simulink model "open_loop_deploy"  (R2026b)
settings: Solver=FixedStepAuto  StopTime=10  EnableMultiTasking=on
undefined symbols (not defined in the file): Bambient, bits, k, R_coil_ref, Vmax
libraries: stm32blockslib x6, stm32f4xxblockslib x1, simulink x1
settings Model: STM32="{\"PWMOutput\":{\"ID\":\"274\"},\"TimerCapture\":[{\"ID\":\"277\"},{\"ID\":\"278\"},{\"ID\":\"279\"},{\"ID\":\"280\"}],\"UARTRead\":{\"ID\":\"339\"},\"UARTWrite\":[{\"ID\":\"366\"},{\"ID\":\"380\"}],\"I2CControllerRead\":{\"ID\":\"388\"},\"I2CControllerWrite\":[{\"ID\":\"398\"},{\"ID\":\"400\"},{\"ID\":\"401\"}]}"  Creator=Samuel  LastModifiedBy=samue
settings SolverCC: AutoInsertRateTranBlk=on
settings OptimizationCC: DefaultParameterBehavior=Inlined  DifferentSizesBufferReuse=on  EfficientTunableParamExpr=on  EnhancedBackFolding=on  MaxStackSize=512  OptimizationCustomize=off  OptimizeBlockOrder=speed  PassReuseOutputArgsAs=Individual arguments  RemoveInternalMemoryZeroInit=on  RemoveRootLevelIOMemoryZeroInit=on
settings DebuggingCC: ParameterTunabilityLossMsg=error
settings HardwareCC: ProdHWDeviceType=ARM Compatible->ARM Cortex-M  ProdLargestAtomicFloat=Double  ProdLargestAtomicInteger=Long  ProdLongLongMode=on
settings SFSimCC: MATLABDynamicMemAlloc=off
settings RTWCC: BuildConfiguration=Faster Runs  Description=Embedded Coder  HardwareBoard=STM32G4xx Based  SystemTargetFile=ert.tlc  TLCOptions=-aInlineSetEventsForThisBaseRateFcn=TLC_FALSE -aSuppressMultiTaskScheduler=TLC_FALSE -aRateBasedStepFcn=1  TemplateMakefile=ert_default_tmf  Toolchain=GNU Tools for STM32
settings CodeAppCC: ForceParamTrailComments=on  IgnoreCustomStorageClasses=off  InsertBlockDesc=on  OperatorAnnotations=on  SFDataObjDesc=on  SimulinkDataObjDesc=on
settings ERTTargetCC: CodeReplacementLibrary=ARM Cortex-M  CombineSignalStateStructs=on  ExtModeIntrfLevel=Level2 - Open  ExtModeMexFile=ext_xcp  ExtModeStaticAlloc=on  SupportVariableSizeSignals=on
settings SimscapeCC: SimscapeUseEnergyAccounting=off

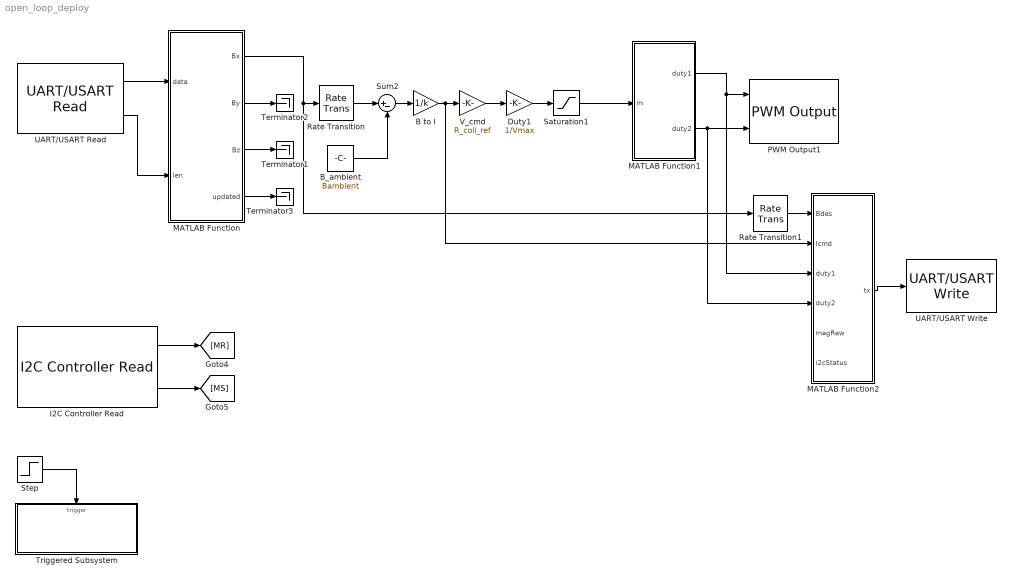
== system open_loop_deploy ==
  B to I : Gain  Gain=1/k
  B_ambient : Constant  Value=Bambient
  Duty1 : Gain  Gain=1/Vmax
  I2C Controller Read : stm32blockslib/I2C Controller Read  I2CModule=I2C1  Mode=Controller  AddressingMode=7-bits  PeripheralByteOrder=BigEndian  OwnPeripheralAddress=uint8(170)  PeripheralAddressVia=Dialog  PeripheralAddress=hex2dec('21')  RegisterAddressMode=on  RegisterAddressVia=Dialog  RegisterAddress=hex2dec('24')  RepeatedStart=off  NoAck=off  OutputStatus=on  BlockMode=Receive  DataType=uint8  DataLength=9  Timeout=0.005  SampleTime=0.01
      settings: LibrarySourceBlock=stm32g4xxblockslib/I2C Controller Read
  MATLAB Function : MATLAB Function  TreatAsAtomicUnit=on
  MATLAB Function1 : MATLAB Function  TreatAsAtomicUnit=on
  MATLAB Function2 : MATLAB Function  TreatAsAtomicUnit=on
  PWM Output1 : stm32f4xxblockslib/PWM Output  ProcessorFamily=STM32G4  TimerModule=TIM1  DutycycleUnits=Percentage  EnableChannel1=on  EnableCaptureCompare1Input=off  EnableCaptureCompare1ComplementaryInput=off  EnableOutputCompare1ModeInput=off  EnableChannel2=on  EnableCaptureCompare2Input=off  EnableCaptureCompare2ComplementaryInput=off  EnableOutputCompare2ModeInput=off  EnableChannel3=off  EnableCaptureCompare3Input=off  EnableCaptureCompare3ComplementaryInput=off  EnableOutputCompare3ModeInput=off  EnableChannel4=off  EnableCaptureCompare4Input=off  EnableCaptureCompare4ComplementaryInput=off  EnableOutputCompare4ModeInput=off  EnableChannel5=off  EnableCaptureCompare5Input=off  EnableOutputCompare5ModeInput=off  EnableChannel6=off  EnableCaptureCompare6Input=off  EnableOutputCompare6ModeInput=off  EnableCounterInput=off  EnableMainOutputInput=off  EnableFrequencyInput=off  SetRCAfterCE=off  OutputDirection=off  OutputMainOutputEnableStatus=off  SampleTime=0.1  EnableSimPort=off  EnableUpdateEvent=off  EnableCaptureCompare1Event=off  EnableCaptureCompare2Event=off  EnableCaptureCompare3Event=off  EnableCaptureCompare4Event=off  EnableTriggerEvent=off  EnableBreakEvent=off  EnableBreakEvent2=off  hoistedMaskSrc=ECSoC/ECSimCodegen/PWM Output
      settings: LibrarySourceBlock=stm32g4xxblockslib/PWM Output
  Rate Transition : RateTransition  OutPortSampleTime=0.1
  Rate Transition1 : RateTransition  OutPortSampleTime=0.1
  Saturation1 : Saturate  UpperLimit=1  LowerLimit=-1
  Step : Step  Time=0.1  SampleTime=0.1
  Sum2 : Sum  Inputs=|+-
  Terminator1 : Terminator
  Terminator2 : Terminator
  Terminator3 : Terminator
  Triggered Subsystem : Subsystem  TreatAsAtomicUnit=on
  UART/USART Read : stm32blockslib/UART//USART Read  UARTModule=LPUART1  DataType=uint8  DataLength=32  BlockingMode=off  BlockingTimeout=0.1  OutputLength=on  OutputStatus=off  SampleTime=0.001
  UART/USART Write : stm32blockslib/UART//USART Write  UARTModule=LPUART1  LengthOfDataToSend=off  BlockingMode=off  BlockingTimeout=0.1  OutputStatus=off
  V_cmd : Gain  Gain=R_coil_ref
  wires:
  B_ambient/1 -> Sum2/2
  Sum2/1 -> B to I/1
  Saturation1/1 -> MATLAB Function1/1(m)
  Duty1/1 -> Saturation1/1
  V_cmd/1 -> Duty1/1
  UART/USART Read/1 -> MATLAB Function/1(data)
  MATLAB Function/3(Bz) -> Terminator1/1
  MATLAB Function/2(By) -> Terminator2/1
  Rate Transition/1 -> Sum2/1
  MATLAB Function/1(Bx) -> Rate Transition/1, Rate Transition1/1
  UART/USART Read/2 -> MATLAB Function/2(len)
  MATLAB Function/4(updated) -> Terminator3/1
  MATLAB Function2/1(tx) -> UART/USART Write/1
  B to I/1 -> MATLAB Function2/2(Icmd), V_cmd/1
  MATLAB Function1/1(duty1) -> MATLAB Function2/3(duty1), PWM Output1/1
  Rate Transition1/1 -> MATLAB Function2/1(Bdes)
  MATLAB Function1/2(duty2) -> MATLAB Function2/4(duty2), PWM Output1/2
  I2C Controller Read/1 -> [MR]
  I2C Controller Read/2 -> [MS]
  Step/1 -> Triggered Subsystem/Trigger

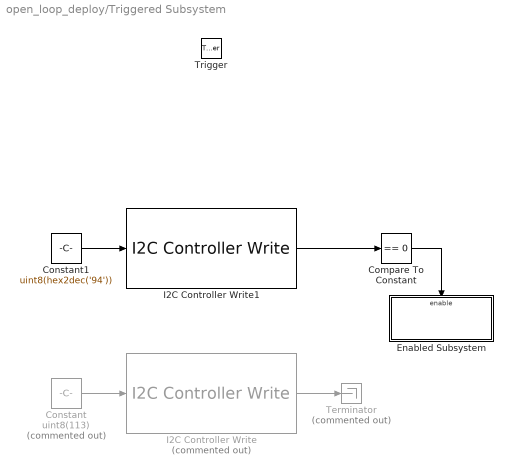
== system open_loop_deploy/Triggered Subsystem ==
  Trigger : TriggerPort  VariantControl=(inherit)
  Compare To Constant : simulink/Logic and Bit Operations/Compare To Constant  relop===  const=0  OutDataTypeStr=boolean
  Constant : Constant  Commented=on  Value=uint8(113)
  Constant1 : Constant  Value=uint8(hex2dec('94'))
  Enabled Subsystem : Subsystem  TreatAsAtomicUnit=on
  I2C Controller Write : stm32blockslib/I2C Controller Write  Commented=on  I2CModule=I2C1  Mode=Controller  AddressingMode=7-bits  PeripheralByteOrder=BigEndian  OwnPeripheralAddress=uint8(170)  PeripheralAddressVia=Dialog  PeripheralAddress=hex2dec('21')  RegisterAddressMode=on  RegisterAddressVia=Dialog  RegisterAddress=1  RepeatedStart=off  NoAck=off  OutputStatus=on  BlockMode=Transmit  DataType=uint8  DataLength=1  Timeout=0.01  SampleTime=-1
      settings: LibrarySourceBlock=stm32g4xxblockslib/I2C Controller Write
  I2C Controller Write1 : stm32blockslib/I2C Controller Write  I2CModule=I2C1  Mode=Controller  AddressingMode=7-bits  PeripheralByteOrder=BigEndian  OwnPeripheralAddress=uint8(170)  PeripheralAddressVia=Dialog  PeripheralAddress=hex2dec('21')  RegisterAddressMode=on  RegisterAddressVia=Dialog  RegisterAddress=hex2dec('0B')  RepeatedStart=off  NoAck=off  OutputStatus=on  BlockMode=Transmit  DataType=uint8  DataLength=1  Timeout=0.01  SampleTime=-1
      settings: LibrarySourceBlock=stm32g4xxblockslib/I2C Controller Write
  Terminator : Terminator  Commented=on
  wires:
  Constant1/1 -> I2C Controller Write1/1
  Compare To Constant/1 -> Enabled Subsystem/Enable
  I2C Controller Write/1 -> Terminator/1
  Constant/1 -> I2C Controller Write/1
  I2C Controller Write1/1 -> Compare To Constant/1

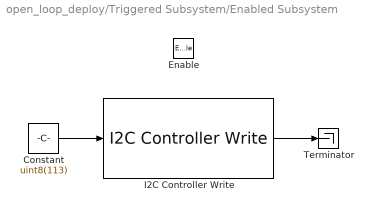
== system open_loop_deploy/Triggered Subsystem/Enabled Subsystem ==
  Enable : EnablePort
  Constant : Constant  Value=uint8(113)
  I2C Controller Write : stm32blockslib/I2C Controller Write  I2CModule=I2C1  Mode=Controller  AddressingMode=7-bits  PeripheralByteOrder=BigEndian  OwnPeripheralAddress=uint8(170)  PeripheralAddressVia=Dialog  PeripheralAddress=hex2dec('21')  RegisterAddressMode=on  RegisterAddressVia=Dialog  RegisterAddress=1  RepeatedStart=off  NoAck=off  OutputStatus=on  BlockMode=Transmit  DataType=uint8  DataLength=1  Timeout=0.01  SampleTime=-1
      settings: LibrarySourceBlock=stm32g4xxblockslib/I2C Controller Write
  Terminator : Terminator
  wires:
  Constant/1 -> I2C Controller Write/1
  I2C Controller Write/1 -> Terminator/1

== matlab function open_loop_deploy/MATLAB Function1 ==
  data: m input; duty1 output; duty2 output
function [duty1, duty2] = drv8871PWM(m)
%#codegen
% m is the normalized voltage command, between -1 and +1.

if m >= 0
    duty1 = 100;
    duty2 = 100 * (1 - m);
else
    duty1 = 100 * (1 + m);
    duty2 = 100;
end

== matlab function open_loop_deploy/MATLAB Function ==
  data: data input; Bx output; len input; By output; Bz output; updated output
function [Bx, By, Bz, updated] = Decode_SET(data, len)
%#codegen
% data: uint8 vector from UART Read, len: number of valid bytes this step.
% GUI sends "SET: x, y, z\n" in microtesla.
persistent buffer count dropping lastB
if isempty(count)
    buffer   = zeros(1, 96, 'uint8');
    count    = 0;
    dropping = false;
    lastB    = zeros(3, 1);
end
updated = false;
nValid = min(double(len), numel(data));
for i = 1:nValid
    b = uint8(data(i));
    if b == 10                          % newline: end of command
        if ~dropping && count > 0
            [vals, ok] = parseSET(buffer, count);
            if ok
                lastB   = vals * 1e-6;  % microtesla -> tesla
                updated = true;
            end
        end
        count    = 0;
        dropping = false;
    elseif b ~= 13                      % ignore carriage return
        if ~dropping
            if count < 96
                count = count + 1;
                buffer(count) = b;
            else
                dropping = true;        % discard oversized line
            end
        end
    end
end
Bx = lastB(1);
By = lastB(2);
Bz = lastB(3);
end

function [vals, ok] = parseSET(buf, n)
vals = zeros(3, 1);
ok = false;
if n < 4
    return;
end
if buf(1) ~= 83 || buf(2) ~= 69 || buf(3) ~= 84 || buf(4) ~= 58   % 'SET:'
    return;
end
pos = 5;
for k = 1:3
    pos = skipSpaces(buf, pos, n);
    if k > 1
        if pos > n || buf(pos) ~= 44    % ','
            return;
        end
        pos = skipSpaces(buf, pos + 1, n);
    end
    [v, pos, good] = parseNum(buf, pos, n);
    if ~good
        return;
    end
    vals(k) = v;
end
pos = skipSpaces(buf, pos, n);
ok = (pos > n);                         % nothing left over
end

function p = skipSpaces(buf, p, n)
while p <= n && (buf(p) == 32 || buf(p) == 9)
    p = p + 1;
end
end

function [v, p, ok] = parseNum(buf, p, n)
v = 0; ok = false; sgn = 1;
if p <= n && (buf(p) == 45 || buf(p) == 43)        % '-' or '+'
    if buf(p) == 45
        sgn = -1;
    end
    p = p + 1;
end
mant = 0; nd = 0;
while p <= n && buf(p) >= 48 && buf(p) <= 57       % integer digits
    mant = mant * 10 + (double(buf(p)) - 48);
    nd = nd + 1; p = p + 1;
end
if p <= n && buf(p) == 46                          % '.'
    p = p + 1; scale = 0.1;
    while p <= n && buf(p) >= 48 && buf(p) <= 57
        mant = mant + (double(buf(p)) - 48) * scale;
        scale = scale / 10;
        nd = nd + 1; p = p + 1;
    end
end
if nd == 0
    return;
end
if p <= n && (buf(p) == 101 || buf(p) == 69)       % 'e' or 'E'
    q = p + 1; esgn = 1;
    if q <= n && (buf(q) == 45 || buf(q) == 43)
        if buf(q) == 45
            esgn = -1;
        end
        q = q + 1;
    end
    ex = 0; ne = 0;
    while q <= n && buf(q) >= 48 && buf(q) <= 57
        ex = ex * 10 + (double(buf(q)) - 48);
        ne = ne + 1; q = q + 1;
    end
    if ne == 0
        return;
    end
    mant = mant * 10^(esgn * ex);
    p = q;
end
v = sgn * mant;
ok = true;
end

== matlab function open_loop_deploy/MATLAB Function2 ==
  data: Bdes input; tx output; Icmd input; duty1 input; duty2 input; magRaw input; i2cStatus input
function tx = Encode_CMD(Bdes, Icmd, duty1, duty2, magRaw, i2cStatus)
%#codegen

values = [double(Bdes)*1e6, double(Icmd), ...
          double(duty1), double(duty2)];

tx = repmat(uint8(32), 1, 80);
tx(1:5) = uint8('CMD: ');
p = 6;

for k = 1:4
    [field, n] = compactNumber(values(k));
    tx(p:p+n-1) = field(1:n);
    p = p + n;
    if k < 4
        tx(p) = uint8(',');
    else
        tx(p) = uint8(10);
    end
    p = p + 1;
end

tx(p:p+4) = uint8('MAG: ');
p = p + 5;

if i2cStatus == 0
    for k = 1:3
        i = 3*(k-1) + 1;
        raw = double(magRaw(i))*65536 ...
            + double(magRaw(i+1))*256 ...
            + double(magRaw(i+2));
        if raw >= 8388608
            raw = raw - 16777216;
        end

        [field, n] = compactNumber(raw / 75);
        tx(p:p+n-1) = field(1:n);
        p = p + n;
        if k < 3
            tx(p) = uint8(',');
            p = p + 1;
        end
    end
else
    tx(p:p+13) = uint8('FAILED_TO_READ');
    p = p + 14;
    tx(p) = uint8(',');
    p = p + 1;
    s = double(i2cStatus);
    started = false;
    for j = 4:-1:0
        divisor = 10^j;
        digit = floor(s / divisor);
        s = mod(s, divisor);
        if digit ~= 0 || started || j == 0
            tx(p) = uint8(digit) + uint8(48);
            p = p + 1;
            started = true;
        end
    end
end

tx(80) = uint8(10);
end

function [out, n] = compactNumber(v)
out = zeros(1, 9, 'uint8');
n = 0;

if ~isfinite(v) || abs(v) > 9999.999
    out(:) = uint8('OVERRANGE');
    n = 9;
    return;
end

q = round(abs(v)*1000);
if v < 0 && q ~= 0
    n = n + 1;
    out(n) = uint8('-');
end

whole = floor(q/1000);
frac = mod(q,1000);
started = false;
for j = 3:-1:0
    divisor = 10^j;
    digit = floor(whole / divisor);
    whole = mod(whole, divisor);
    if digit ~= 0 || started || j == 0
        n = n + 1;
        out(n) = uint8(digit) + uint8(48);
        started = true;
    end
end

if frac ~= 0
    n = n + 1;
    out(n) = uint8('.');
    for j = 2:-1:0
        divisor = 10^j;
        digit = floor(frac / divisor);
        frac = mod(frac, divisor);
        n = n + 1;
        out(n) = uint8(digit) + uint8(48);
        if frac == 0
            break;
        end
    end
end
end
